simulink model "sf_temporalcount_indexing_vector"  (R2025b)
settings: Solver=FixedStepDiscrete  StartTime=0.0  StopTime=100  FixedStep=0.5  RelTol=1e-3  EnableMultiTasking=on
settings Model: Creator=The MathWorks, Inc.  LastModifiedBy=The MathWorks, Inc.
settings SolverCC: AlgebraicLoopSolver=TrustRegion
settings DataIOCC: LimitDataPoints=on  SaveFormat=Array  ReturnWorkspaceOutputs=off
settings OptimizationCC: ReuseModelBlockBuffer=off  ExpressionDepthLimit=2147483647.0  InitFltsAndDblsToZero=on  LifeSpan=inf
settings DebuggingCC: UnderspecifiedInitializationDetection=Classic  MergeDetectMultiDrivingBlocksExec=none  SolverPrmCheckMsg=warning  FcnCallInpInsideContextMsg=warning  UnconnectedInputMsg=warning  UnconnectedOutputMsg=warning  UnconnectedLineMsg=warning  StateNameClashWarn=warning  SFUnexpectedBacktrackingDiag=warning  SFNoUnconditionalDefaultTransitionDiag=warning  SFExecutionAtInitializationDiag=none  ArithmeticOperatorsInVariantConditions=warning
settings HardwareCC: ProdBitPerPointer=32.0  ProdBitPerSizeT=32.0  ProdBitPerPtrDiffT=32.0  ProdLargestAtomicFloat=None  ProdIntDivRoundTo=Undefined  ProdEndianess=Unspecified  ProdWordSize=32.0  ProdHWDeviceType=32-bit Generic
settings ModelReferenceCC: EnableRefExpFcnMdlSchedulingChecks=on  PropagateSignalLabelsOutOfModel=off
settings SFSimCC: SimUseLocalCustomCode=off  SimParseCustomCode=off  CustomCodeUndefinedFunction=UseInterfaceOnly
settings RTWCC: RTWUseLocalCustomCode=off  GPUComputeCapability=3.5
settings CodeAppCC: StateflowObjectComments=on
settings GRTTargetCC: TargetLangStandard=C89/C90 (ANSI)  CombineOutputUpdateFcns=off  GRTInterface=on
settings ConfigComp: CovMetricSettings=dw  CovSaveCumulativeToWorkspaceVar=on  CovSaveSingleToWorkspaceVar=on  CovExternalEMLEnable=off

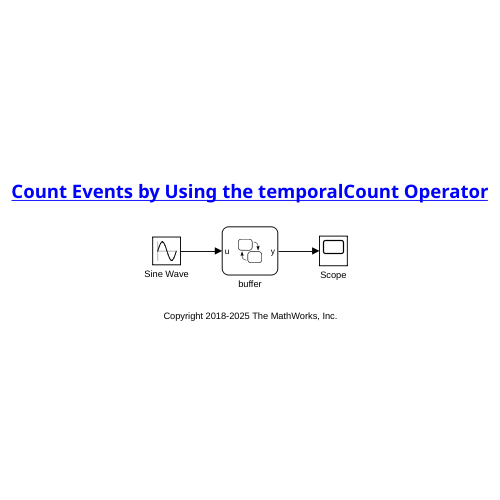
[thumbnail: Simulink's stored preview of the top-level diagram]
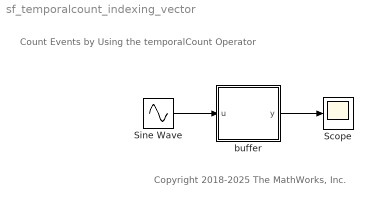
== system sf_temporalcount_indexing_vector ==
  note: Copyright 2018-2025 The MathWorks, Inc.
  note: Count Events by Using the temporalCount Operator
  Scope : Scope
  Sine Wave : Sin  Amplitude=10  Bias=10  Frequency=0.1  SampleTime=0
  buffer : Stateflow chart  TreatAsAtomicUnit=on
  wires:
  buffer/1(y) -> Scope/1
  Sine Wave/1 -> buffer/1(u)

== stateflow chart sf_temporalcount_indexing_vector/buffer ==
  state Observe
  state Collect_Data
    // store first element
    entry: y[0] = u;
    // index values into vector
    during: y[temporalCount(tick)] = u;
    // print values upon exit
    exit: status()
  (default) -> Observe
  Observe -> Collect_Data : [u > 0]
  Collect_Data -> Observe : after(10, tick)
  data: u input; y output double size=10
  function status:
    | function status()
    | %#codegen
    | coder.extrinsic('disp');
    | 
    | % Add separator between buffer dumps
    | persistent alreadyRan
    | 
    | if isempty(alreadyRan)
    |     alreadyRan = true;
    | else
    |     disp('----------');
    | end
    | 
    | % Display the values in the buffer array
    | disp(y);
